simulink model "CSE_project"  (R2024a)
settings: Solver=FixedStepAuto  StartTime=0.0  StopTime=100  FixedStep=0.02  RelTol=1e-3  EnableMultiTasking=on
libraries: dspstat3 x1, slpidlib x1, arduinolib x1, arduinosensorlib x1
settings Model: ExtModeTrigDuration=2  Creator=aksha  LastModifiedBy=aksha
settings SolverCC: AutoInsertRateTranBlk=on
settings OptimizationCC: EnhancedBackFolding=on  PassReuseOutputArgsAs=Individual arguments  ZeroExternalMemoryAtStartup=off  ZeroInternalMemoryAtStartup=off  MaxStackSize=64  OptimizeBlockOrder=speed  DifferentSizesBufferReuse=on  EfficientTunableParamExpr=on
settings DebuggingCC: ParameterTunabilityLossMsg=error
settings HardwareCC: ProdBitPerInt=16  ProdBitPerPointer=16  ProdBitPerSizeT=16  ProdBitPerPtrDiffT=16  ProdLargestAtomicFloat=None  ProdWordSize=8  ProdHWDeviceType=Atmel->AVR
settings SFSimCC: MATLABDynamicMemAlloc=off
settings RTWCC: Description=Embedded Coder  SystemTargetFile=ert.tlc  HardwareBoard=Arduino Uno  TemplateMakefile=ert_default_tmf  Toolchain=Arduino AVR  BuildConfiguration=Faster Runs
settings CodeAppCC: ForceParamTrailComments=on  IgnoreCustomStorageClasses=off  OperatorAnnotations=on  SimulinkDataObjDesc=on  SFDataObjDesc=on  InsertBlockDesc=on
settings ERTTargetCC: SupportContinuousTime=on  SupportVariableSizeSignals=on  ExtMode=on  ExtModeTransport=3  ExtModeStaticAlloc=on  ExtModeAutomaticAllocSize=off  ExtModeStaticAllocSize=250  ExtModeMexFile=ext_xcp  ExtModeMexArgs=1 14 115200  ExtModeIntrfLevel=Level2 - Open

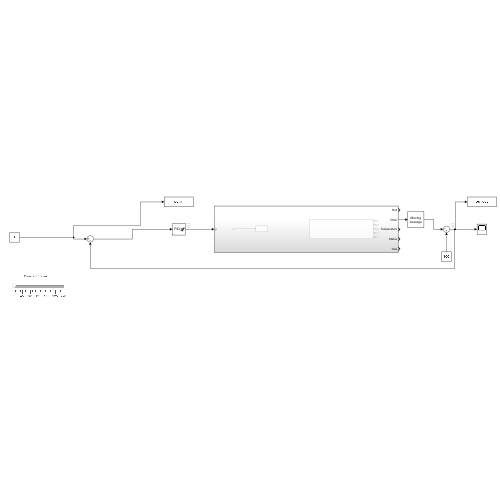
[thumbnail: Simulink's stored preview of the top-level diagram]
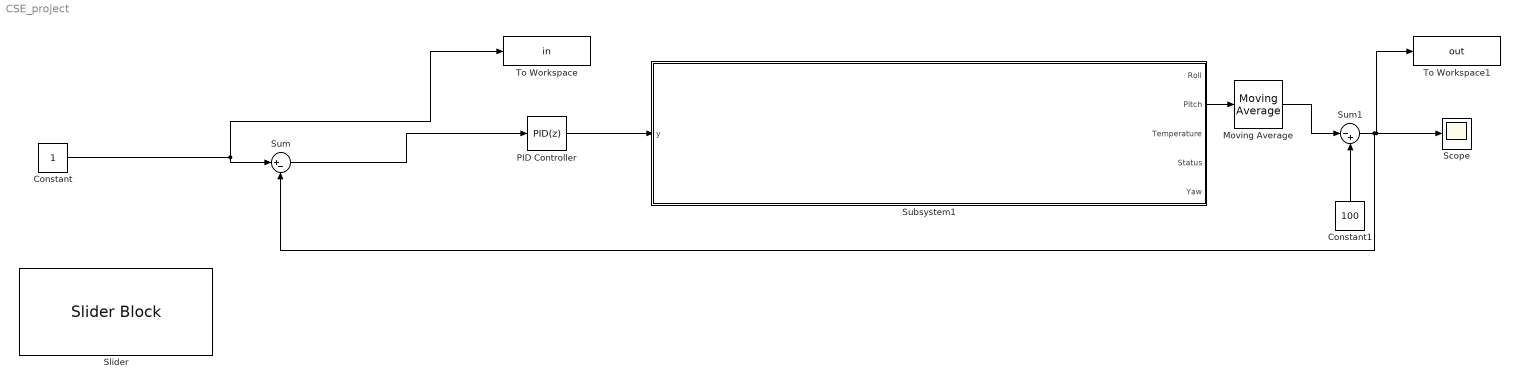
== system CSE_project ==
  Constant : Constant
  Constant1 : Constant  Value=100
  Moving Average : dspstat3/Moving Average  Method=Sliding window  ForgettingFactorPort=off  SpecifyWindowLength=on  WindowLength=4  OverlapLength=3  AllowArbitraryInputLength=off  ForgettingFactor=0.9  SimulateUsing=Interpreted execution
  PID Controller : slpidlib/PID Controller  Controller=PID  Form=Ideal  TimeDomain=Discrete-time  UseExternalTs=off  SampleTime=-1  IntegratorMethod=Forward Euler  FilterMethod=Forward Euler  ControllerParametersSource=internal  P=500  I=300  UseKiTs=off  D=0.01  UseExternalDerivativeSource=off  N=100  UseFilter=on  TunerSelectOption=Transfer Function Based (PID Tuner App)  InitialConditionSource=internal  InitialConditionForIntegrator=95  InitialConditionForFilter=95  DifferentiatorICPrevScaledInput=0  ExternalReset=none  TrackingMode=off  Kt=1  LimitOutput=on  SatLimitsSource=internal  UpperSaturationLimit=118  LowerSaturationLimit=95  LinearizeAsGain=on  AntiWindupMode=clamping  Kb=1  LimitIntegrator=off  UpperIntegratorSaturationLimit=inf  LowerIntegratorSaturationLimit=-inf  POutMin=[]  POutMax=[]  IOutMin=[]  IOutMax=[]  DOutMin=[]  DOutMax=[]  NOutMin=[]  NOutMax=[]  SumOutMin=[]  SumOutMax=[]  SaturationOutMin=[]  SaturationOutMax=[]  PParamMin=[]  PParamMax=[]  IParamMin=[]  IParamMax=[]  DParamMin=[]  DParamMax=[]  NParamMin=[]  NParamMax=[]  KbParamMin=[]  KbParamMax=[]  KtParamMin=[]  KtParamMax=[]  KbOutMin=[]  KbOutMax=[]  KtOutMin=[]  KtOutMax=[]  IntegratorOutMin=[]  IntegratorOutMax=[]  FilterOutMin=[]  FilterOutMax=[]  SumI1OutMin=[]  SumI1OutMax=[]  SumI2OutMin=[]  SumI2OutMax=[]  SumI3OutMin=[]  SumI3OutMax=[]  SumI4OutMin=[]  SumI4OutMax=[]  SumDOutMin=[]  SumDOutMax=[]  DifferentiatorOutMin=[]  DifferentiatorOutMax=[]  FilterDiffOutCoefMin=[]  FilterDiffOutCoefMax=[]  ReciprocalOutMin=[]  ReciprocalOutMax=[]  SumDenOutMin=[]  SumDenOutMax=[]  SumNumOutMin=[]  SumNumOutMax=[]  DivideOutMin=[]  DivideOutMax=[]  UdiffTsProdOutMin=[]  UdiffTsProdOutMax=[]  NTsProdOutMin=[]  NTsProdOutMax=[]  UintegralTsProdOutMin=[]  UintegralTsProdOutMax=[]  UngainTsProdOutMin=[]  UngainTsProdOutMax=[]  ClampingZeroOutDataTypeStr=Inherit: Inherit via back propagation  ClampingZeroOutMin=[]  ClampingZeroOutMax=[]  FilterDenConstantOutDataTypeStr=Inherit: Inherit via back propagation  FilterDenConstantOutMin=[]  FilterDenConstantOutMax=[]  PCopyOutDataTypeStr=Inherit: Inherit via back propagation  PCopyOutMin=[]  PCopyOutMax=[]  NCopyOutDataTypeStr=Inherit: Inherit via back propagation  NCopyOutMin=[]  NCopyOutMax=[]  IntegratorContinuousStateAttributes=''  IntegratorStateMustResolveToSignalObject=off  IntegratorRTWStateStorageClass=Auto  FilterContinuousStateAttributes=''  FilterStateMustResolveToSignalObject=off  FilterRTWStateStorageClass=Auto  ParallelPVariant=Passthrough  IdealPVariant=InternalParameters  IVariant=InternalParameters  DVariant=InternalParameters  IntegratorVariant=Discrete  SatVariant=Enabled  AWVariant=DiscClampingIdeal  PCopyVariant=InternalParamsIdeal  TRVariant=Disabled  FdbkBlocksVariant=Forward  IdealPFdbkVariant=Disabled  SatFdbkVariant=Disabled  DerivativeFilterVariant=ForwardEulerFilter  NVariant=InternalParameters  NCopyVariant=Disabled  FilterICVariant=InternalICsFilter  IntegratorICVariant=InternalICs  ExternalResetVariant=Disabled  TRSumVariant=Passthrough  SumFdbkVariant=Disabled  SumVariant=Sum_PID  TsampFilterVariant=InternalTs  TsampNgainVariant=Passthrough  TsampIntegralVariant=Disabled_SignalSpec  ExternalSaturationOutDataTypeStr=Inherit: Same as second input  DerivativeSourceVariant=ErrorSignal
  Scope : Scope
  Slider : SliderBlock  ScaleMax=270
  Subsystem1 : Subsystem
  Sum : Sum  Inputs=|+-
  Sum1 : Sum  Inputs=|-+
  To Workspace : ToWorkspace  VariableName=in  SaveFormat=Timeseries  SampleTime=-1
  To Workspace1 : ToWorkspace  VariableName=out  SaveFormat=Timeseries  SampleTime=-1
  wires:
  Sum/1 -> PID Controller/1
  Subsystem1/2(Pitch) -> Moving Average/1
  Constant1/1 -> Sum1/2
  Sum1/1 -> Scope/1, To Workspace1/1, Sum/2
  Moving Average/1 -> Sum1/1
  PID Controller/1 -> Subsystem1/1(y)
  Constant/1 -> Sum/1, To Workspace/1

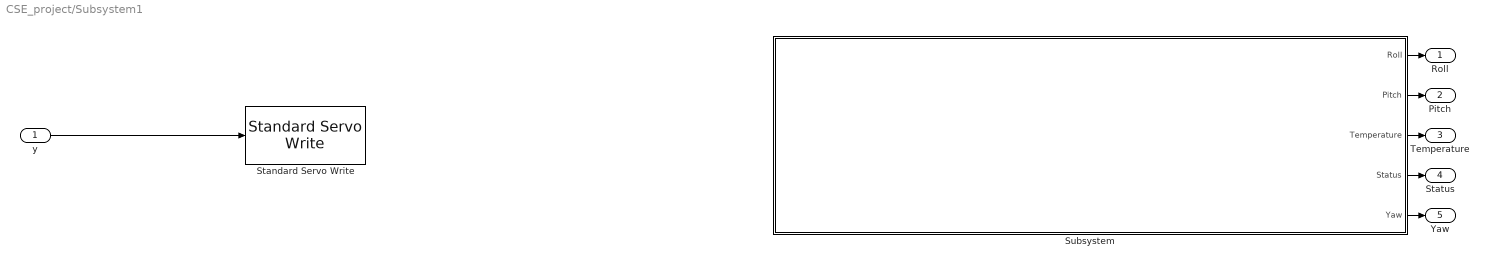
== system CSE_project/Subsystem1 ==
  y : Inport
  Standard Servo Write : arduinolib/Standard Servo Write  pinNumber=9  ServoIndex=0  blockPlatform=ARDUINO
      settings: SourceProductName=Common
  Subsystem : Subsystem
  Roll : Outport
  Pitch : Outport  Port=2
  Temperature : Outport  Port=3
  Status : Outport  Port=4
  Yaw : Outport  Port=5
  wires:
  Subsystem/2(Pitch) -> Pitch/1
  Subsystem/1(Roll) -> Roll/1
  Subsystem/3(Temperature) -> Temperature/1
  y/1 -> Standard Servo Write/1
  Subsystem/4(Status) -> Status/1
  Subsystem/5(Yaw) -> Yaw/1

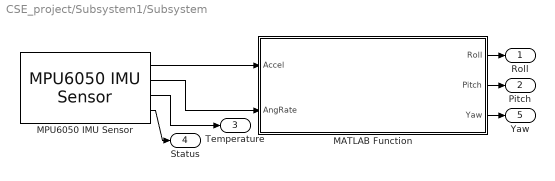
== system CSE_project/Subsystem1/Subsystem ==
  MATLAB Function : MATLAB Function  TreatAsAtomicUnit=on
  MPU6050 IMU Sensor : arduinosensorlib/MPU6050 IMU Sensor  I2CModule=0  SlaveAddress=0x68  Accel=on  AngularRate=on  Temperature=on  Status=on  Timestamp=off  EulerAngles=off  Quat=off  AccelRange=2G  GyroRange=250 dps  DmpOdr=200 Hz  Dlpf=Accelerometer: 94Hz, Gyroscope: 98Hz  spf=1  SampleTime=-1  QueueSizeFactor=1
      settings: SourceProductName=Sensors
  Roll : Outport
  Pitch : Outport  Port=2
  Temperature : Outport  Port=3
  Status : Outport  Port=4
  Yaw : Outport  Port=5
  wires:
  MPU6050 IMU Sensor/3 -> Temperature/1
  MATLAB Function/1(Roll) -> Roll/1
  MPU6050 IMU Sensor/1 -> MATLAB Function/1(Accel)
  MPU6050 IMU Sensor/2 -> MATLAB Function/2(AngRate)
  MPU6050 IMU Sensor/4 -> Status/1
  MATLAB Function/2(Pitch) -> Pitch/1
  MATLAB Function/3(Yaw) -> Yaw/1

== matlab function CSE_project/Subsystem1/Subsystem/MATLAB Function ==
  data: Accel input; Roll output; AngRate input; Pitch output; Yaw output

function [Roll, Pitch, Yaw] = attitude(Accel, AngRate)

% Lightweight scalar Kalman filter
% Sampling frequency = 50 Hz

persistent roll pitch yaw
persistent Pr Pp

Ts = single(0.02);

Q = single(0.001);
R = single(0.03);

if isempty(roll)

    ax = single(Accel(1));
    ay = single(Accel(2));
    az = single(Accel(3));

    roll = atan2(ay,az);

    pitch = atan2(-ax,sqrt(ay*ay + az*az));

    yaw = single(0);

    Pr = single(1);
    Pp = single(1);

end

% Accelerometer measurements
ax = single(Accel(1));
ay = single(Accel(2));
az = single(Accel(3));

accRoll = atan2(ay,az);

accPitch = atan2(-ax,sqrt(ay*ay + az*az));

% Gyroscope measurements
gx = single(AngRate(1))*single(0.017453293);
gy = single(AngRate(2))*single(0.017453293);
gz = single(AngRate(3))*single(0.017453293);

% ROLL FILTER
rollPred = roll + gx*Ts;

Pr = Pr + Q;

Kr = Pr/(Pr+R);

roll = rollPred + Kr*(accRoll-rollPred);

Pr = (single(1)-Kr)*Pr;

% PITCH FILTER
pitchPred = pitch + gy*Ts;

Pp = Pp + Q;

Kp = Pp/(Pp+R);

pitch = pitchPred + Kp*(accPitch-pitchPred);

Pp = (single(1)-Kp)*Pp;

% YAW
yaw = yaw + gz*Ts;

% Output in degrees
Roll = roll*single(57.29578);
Pitch = pitch*single(57.29578);
Yaw = yaw*single(57.29578);

end
